simulink model "CIFB4"  (R2022b)
settings: Solver=FixedStepDiscrete  StartTime=0.0  StopTime=0.01  RelTol=1e-3
libraries: dspsrcs4 x1
settings Model: Creator=ASAA  LastModifiedBy=ASAA

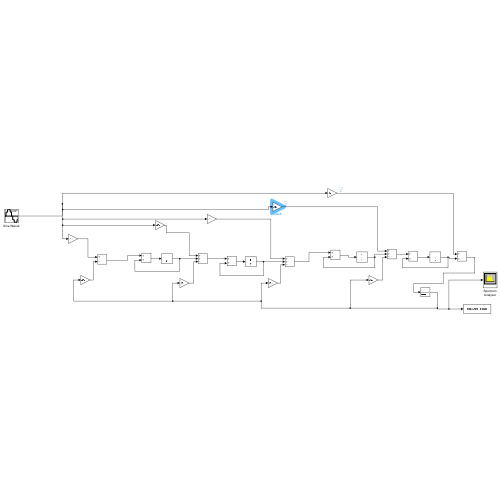
[thumbnail: Simulink's stored preview of the top-level diagram]
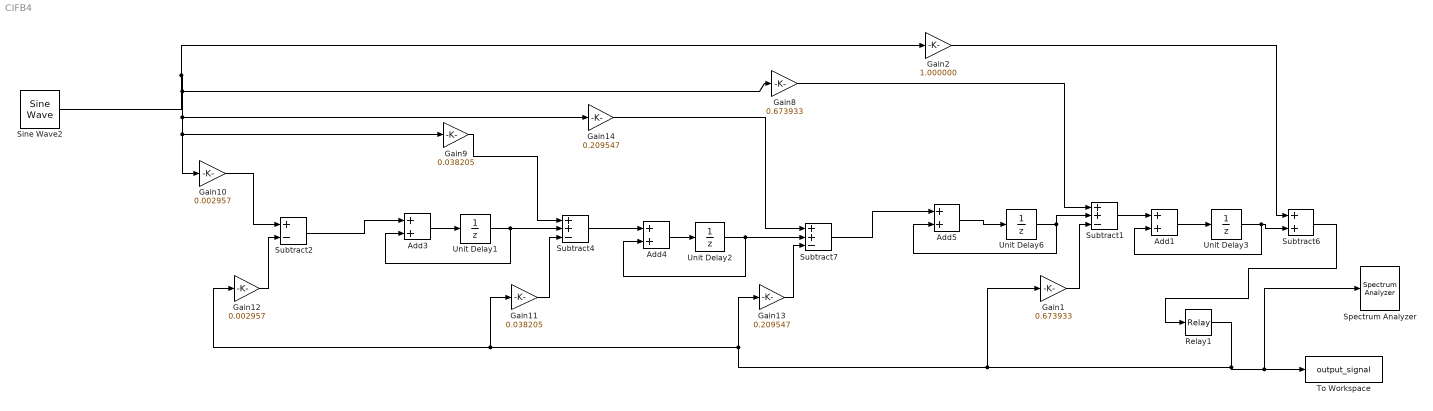
== system CIFB4 ==
  Add{1,3..5} (4 alike) : Sum
  Gain1 : Gain  Gain=0.673933
  Gain10 : Gain  Gain=0.002957
  Gain11 : Gain  Gain=0.038205
  Gain12 : Gain  Gain=0.002957
  Gain13 : Gain  Gain=0.209547
  Gain14 : Gain  Gain=0.209547
  Gain2 : Gain  Gain=1.000000
  Gain8 : Gain  Gain=0.673933
  Gain9 : Gain  Gain=0.038205
  Relay1 : Relay  OffOutputValue=-1
  Sine Wave2 : dspsrcs4/Sine Wave  Amplitude=0.63  Frequency=100e3  Phase=0  SampleMode=Discrete  OutComplex=Real  CompMethod=Trigonometric fcn  TableSize=Speed  SampleTime=1e-8  SamplesPerFrame=1  ResetState=Restart at time zero  OutputFrames=off  dataType=double  wordLen=16  udDataType=sfix(16)  fracBitsMode=Best precision  numFracBits=15  OutDataTypeStr=double  LastOutDataTypeStr=double
  Spectrum Analyzer : SpectrumAnalyzer
  Subtract1 : Sum  Inputs=++-
  Subtract2 : Sum  Inputs=+-
  Subtract4 : Sum  Inputs=++-
  Subtract6 : Sum
  Subtract7 : Sum  Inputs=++-
  To Workspace : ToWorkspace  VariableName=output_signal  SaveFormat=Timeseries  SampleTime=-1
  Unit Delay{1..3,6} (4 alike) : UnitDelay  SampleTime=1/100e6  HasFrameUpgradeWarning=on
  wires:
  Subtract4/1 -> Add4/1
  Gain14/1 -> Subtract7/1
  Subtract6/1 -> Relay1/1
  Add4/1 -> Unit Delay2/1
  Add3/1 -> Unit Delay1/1
  Gain13/1 -> Subtract7/3
  Unit Delay2/1 -> Subtract7/2, Add4/2
  Unit Delay1/1 -> Subtract4/2, Add3/2
  Gain9/1 -> Subtract4/1
  Gain10/1 -> Subtract2/1
  Gain11/1 -> Subtract4/3
  Relay1/1 -> Gain1/1, Gain12/1, Gain11/1, Gain13/1, Spectrum Analyzer/1, To Workspace/1
  Gain12/1 -> Subtract2/2
  Subtract2/1 -> Add3/1
  Sine Wave2/1 -> Gain2/1, Gain8/1, Gain14/1, Gain9/1, Gain10/1
  Add5/1 -> Unit Delay6/1
  Unit Delay6/1 -> Subtract1/2, Add5/2
  Subtract7/1 -> Add5/1
  Gain8/1 -> Subtract1/1
  Gain1/1 -> Subtract1/3
  Gain2/1 -> Subtract6/1
  Add1/1 -> Unit Delay3/1
  Subtract1/1 -> Add1/1
  Unit Delay3/1 -> Add1/2, Subtract6/2
